simulink model "WindPVStorage_AC_Island"  (R2025a)
settings: Solver=FixedStepDiscrete  StartTime=0.0  StopTime=48  FixedStep=1e-4  RelTol=1e-3
libraries: spsGroundLib x9, spsControlledCurrentSourceLib x6, spsThreePhaseParallelRLCLoadLib x5, spsThreePhaseVIMeasurementLib x5, spsSeriesRLCBranchLib x3, spsControlledVoltageSourceLib x3, spsThreePhaseBreakerLib x3, spspowerguiLib x1
settings Model: Creator=cherrycai  LastModifiedBy=cherrycai
settings DataIOCC: SaveOutput=off  SaveTime=off

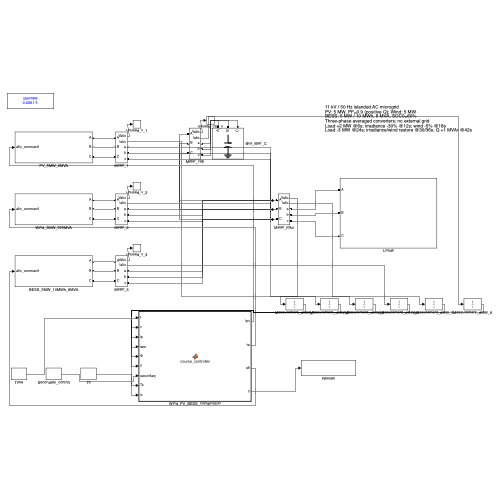
[thumbnail: Simulink's stored preview of the top-level diagram]
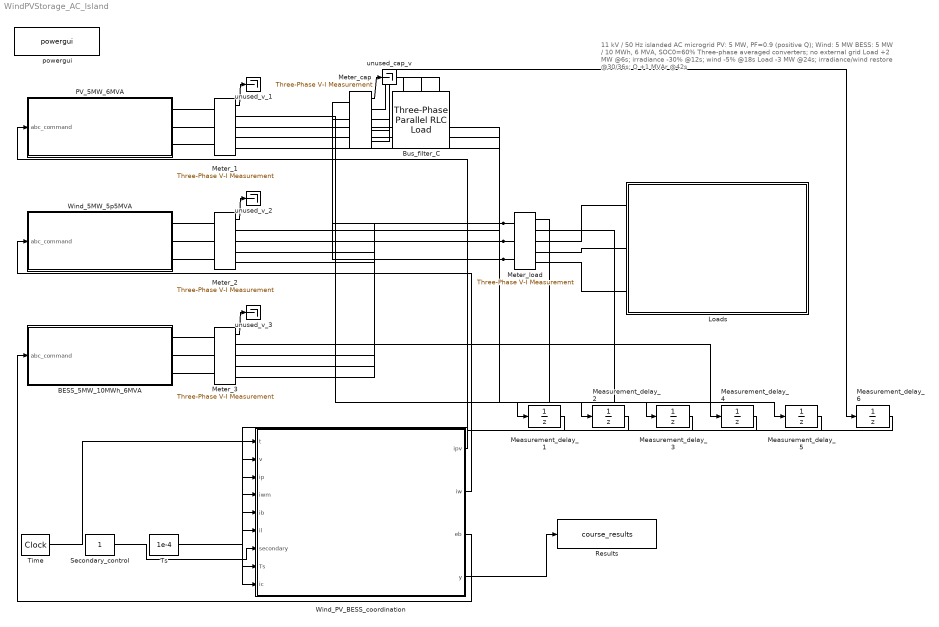
== system WindPVStorage_AC_Island ==
  note: 11 kV / 50 Hz islanded AC microgrid
      | PV: 5 MW, PF=0.9 (positive Q); Wind: 5 MW
      | BESS: 5 MW / 10 MWh, 6 MVA, SOC0=60%
      | Three-phase averaged converters; no external grid
      | Load +2 MW @6s; irradiance -30% @12s; wind -5% @18s
      | Load -3 MW @24s; irradiance/wind restore @30/36s; Q +1 MVAr @42s
  BESS_5MW_10MWh_6MVA : Subsystem
  Bus_filter_C : spsThreePhaseParallelRLCLoadLib/Three-Phase Parallel RLC Load  LConnTagsString=A|B|C  Configuration=Y (grounded)  NominalVoltage=11000  Vabc=[1e3 1e3 1e3]  Vabcp=[1e3 1e3 1e3]  NominalFrequency=50  UnbalancedPower=off  ActivePower=0  InductivePower=0  CapacitivePower=2e5  Pabc=[10e3 9e3 11e3]  QLabc=[100 90 110]  QCabc=[100 90 110]  Pabcp=[10e3 9e3 11e3]  QLabcp=[100 90 110]  QCabcp=[100 90 110]  Measurements=None  LoadType=constant Z
  Loads : Subsystem
  Measurement_delay_{1..6} (6 alike) : UnitDelay  InitialCondition=[0 0 0]  SampleTime=1e-4  HasFrameUpgradeWarning=on
  Meter_1 : spsThreePhaseVIMeasurementLib/Three-Phase V-I Measurement  VoltageMeasurement=phase-to-ground  SetLabelV=off  LabelV=Vabc  Vpu=off  VpuLL=off  CurrentMeasurement=yes  SetLabelI=off  LabelI=Iabc  Ipu=off  Pbase=100e6  Vbase=500e3  OutputType=Complex  PhasorSimulation=off  PSBequivalent=0
  Meter_2 : spsThreePhaseVIMeasurementLib/Three-Phase V-I Measurement  VoltageMeasurement=phase-to-ground  SetLabelV=off  LabelV=Vabc  Vpu=off  VpuLL=off  CurrentMeasurement=yes  SetLabelI=off  LabelI=Iabc  Ipu=off  Pbase=100e6  Vbase=500e3  OutputType=Complex  PhasorSimulation=off  PSBequivalent=0
  Meter_3 : spsThreePhaseVIMeasurementLib/Three-Phase V-I Measurement  VoltageMeasurement=phase-to-ground  SetLabelV=off  LabelV=Vabc  Vpu=off  VpuLL=off  CurrentMeasurement=yes  SetLabelI=off  LabelI=Iabc  Ipu=off  Pbase=100e6  Vbase=500e3  OutputType=Complex  PhasorSimulation=off  PSBequivalent=0
  Meter_cap : spsThreePhaseVIMeasurementLib/Three-Phase V-I Measurement  VoltageMeasurement=phase-to-ground  SetLabelV=off  LabelV=Vabc  Vpu=off  VpuLL=off  CurrentMeasurement=yes  SetLabelI=off  LabelI=Iabc  Ipu=off  Pbase=100e6  Vbase=500e3  OutputType=Complex  PhasorSimulation=off  PSBequivalent=0
  Meter_load : spsThreePhaseVIMeasurementLib/Three-Phase V-I Measurement  VoltageMeasurement=phase-to-ground  SetLabelV=off  LabelV=Vabc  Vpu=off  VpuLL=off  CurrentMeasurement=yes  SetLabelI=off  LabelI=Iabc  Ipu=off  Pbase=100e6  Vbase=500e3  OutputType=Complex  PhasorSimulation=off  PSBequivalent=0
  PV_5MW_6MVA : Subsystem
  Results : ToWorkspace  VariableName=course_results  SaveFormat=Timeseries  SampleTime=-1
      settings: Decimation=10
  Secondary_control : Constant
  Time : DigitalClock  SampleTime=1e-4
  Ts : Constant  Value=1e-4
  Wind_5MW_5p5MVA : Subsystem
  Wind_PV_BESS_coordination : MATLAB Function  TreatAsAtomicUnit=on
  powergui : spspowerguiLib/powergui  Priority=1  SimulationMode=Discrete  SampleTime=1e-4  frequency=50  Iterations=50  frequencyindice=50  Pbase=100e6  ErrMax=1e-4  UnitsV=kV  UnitsW=MW  buscounter=0  FunctionMessages=off  echomessages=off  EnableUseOfTLC=off  CurrentSourceSwitches=off  DisableSnubberDevices=off  DisableRonSwitches=off  DisableVfSwitches=off  DisplayEquations=off  AutomaticDiscreteSolvers=off  SolverType=Tustin/Backward Euler (TBE)  Interpol=off  ExternalGateDelay=off  methode=off  Ts=100  x0status=blocks  SPID=on  SwTol=0  HookPort=off  NonlinearTolerance=1e-4  nMaxIteration=100  ContinueOnMaxIteration=off  RestoreLinks=warning  ResistiveCurrentMeasurement=off  Frange=[0:2:500]  Ylog=off  Xlog=on  ShowGrid=off  save=off  variable=ZData  structure=0  ZoomFFT=off  StartTime=0.0  cycles=1  DisplayStyle=1  fundamental=50  FreqAxis=off  MaxFrequency=1000  frequencyindicesteady=1  RmsSteady=1  display=off
  unused_cap_v : Terminator
  unused_v_1 : Terminator
  unused_v_2 : Terminator
  unused_v_3 : Terminator
  wires:
  Time/1 -> Wind_PV_BESS_coordination/1(t)
  Secondary_control/1 -> Wind_PV_BESS_coordination/7(secondary)
  Ts/1 -> Wind_PV_BESS_coordination/8(Ts)
  Wind_PV_BESS_coordination/1(ipv) -> PV_5MW_6MVA/1(abc_command)
  Wind_PV_BESS_coordination/2(iw) -> Wind_5MW_5p5MVA/1(abc_command)
  Wind_PV_BESS_coordination/3(eb) -> BESS_5MW_10MWh_6MVA/1(abc_command)
  Meter_cap/2 -> Measurement_delay_6/1
  Measurement_delay_6/1 -> Wind_PV_BESS_coordination/9(ic)
  Meter_cap/1 -> unused_cap_v/1
  Meter_load/1 -> Measurement_delay_1/1
  Measurement_delay_1/1 -> Wind_PV_BESS_coordination/2(v)
  Meter_1/2 -> Measurement_delay_2/1
  Measurement_delay_2/1 -> Wind_PV_BESS_coordination/3(ip)
  Meter_2/2 -> Measurement_delay_3/1
  Measurement_delay_3/1 -> Wind_PV_BESS_coordination/4(iwm)
  Meter_3/2 -> Measurement_delay_4/1
  Measurement_delay_4/1 -> Wind_PV_BESS_coordination/5(ib)
  Meter_load/2 -> Measurement_delay_5/1
  Measurement_delay_5/1 -> Wind_PV_BESS_coordination/6(il)
  Wind_PV_BESS_coordination/4(y) -> Results/1
  Meter_1/1 -> unused_v_1/1
  Meter_2/1 -> unused_v_2/1
  Meter_3/1 -> unused_v_3/1
  connections:
  PV_5MW_6MVA/RConn1 -- Meter_1/LConn1
  PV_5MW_6MVA/RConn2 -- Meter_1/LConn2
  PV_5MW_6MVA/RConn3 -- Meter_1/LConn3
  Wind_5MW_5p5MVA/RConn1 -- Meter_2/LConn1
  Wind_5MW_5p5MVA/RConn2 -- Meter_2/LConn2
  Wind_5MW_5p5MVA/RConn3 -- Meter_2/LConn3
  BESS_5MW_10MWh_6MVA/RConn1 -- Meter_3/LConn1
  BESS_5MW_10MWh_6MVA/RConn2 -- Meter_3/LConn2
  BESS_5MW_10MWh_6MVA/RConn3 -- Meter_3/LConn3
  Meter_1/RConn1 -- Meter_2/RConn1 -- Meter_3/RConn1 -- Meter_load/LConn1 -- Meter_cap/LConn1
  Meter_1/RConn2 -- Meter_2/RConn2 -- Meter_3/RConn2 -- Meter_load/LConn2 -- Meter_cap/LConn2
  Meter_1/RConn3 -- Meter_2/RConn3 -- Meter_3/RConn3 -- Meter_load/LConn3 -- Meter_cap/LConn3
  Meter_load/RConn1 -- Loads/LConn1
  Meter_load/RConn2 -- Loads/LConn2
  Meter_load/RConn3 -- Loads/LConn3
  Meter_cap/RConn1 -- Bus_filter_C/LConn1
  Meter_cap/RConn2 -- Bus_filter_C/LConn2
  Meter_cap/RConn3 -- Bus_filter_C/LConn3

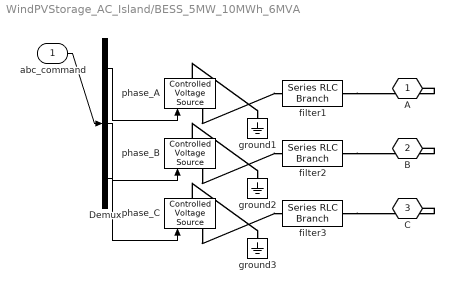
== system WindPVStorage_AC_Island/BESS_5MW_10MWh_6MVA ==
  abc_command : Inport
  Demux : Demux  Outputs=3
  filter1 : spsSeriesRLCBranchLib/Series RLC Branch  LConnTagsString=__new0  RConnTagsString=__new0  BranchType=RL  Resistance=.15  Inductance=.003  SetiL0=off  InitialCurrent=0  Capacitance=1e-6  Setx0=off  InitialVoltage=0  Measurements=None
  filter2 : spsSeriesRLCBranchLib/Series RLC Branch  LConnTagsString=__new0  RConnTagsString=__new0  BranchType=RL  Resistance=.15  Inductance=.003  SetiL0=off  InitialCurrent=0  Capacitance=1e-6  Setx0=off  InitialVoltage=0  Measurements=None
  filter3 : spsSeriesRLCBranchLib/Series RLC Branch  LConnTagsString=__new0  RConnTagsString=__new0  BranchType=RL  Resistance=.15  Inductance=.003  SetiL0=off  InitialCurrent=0  Capacitance=1e-6  Setx0=off  InitialVoltage=0  Measurements=None
  ground1 : spsGroundLib/Ground  LConnTagsString=a
  ground2 : spsGroundLib/Ground  LConnTagsString=a
  ground3 : spsGroundLib/Ground  LConnTagsString=a
  phase_A : spsControlledVoltageSourceLib/Controlled Voltage Source  Initialize=off  Source_Type=AC  Amplitude=0  Phase=0  Frequency=0  Measurements=None
  phase_B : spsControlledVoltageSourceLib/Controlled Voltage Source  Initialize=off  Source_Type=AC  Amplitude=0  Phase=0  Frequency=0  Measurements=None
  phase_C : spsControlledVoltageSourceLib/Controlled Voltage Source  Initialize=off  Source_Type=AC  Amplitude=0  Phase=0  Frequency=0  Measurements=None
  A : PMIOPort  Side=Right
  B : PMIOPort  Port=2  Side=Right
  C : PMIOPort  Port=3  Side=Right
  wires:
  abc_command/1 -> Demux/1
  Demux/1 -> phase_A/1
  Demux/2 -> phase_B/1
  Demux/3 -> phase_C/1
  connections:
  phase_A/RConn1 -- ground1/LConn1
  phase_A/LConn1 -- filter1/LConn1
  filter1/RConn1 -- A/RConn1
  phase_B/RConn1 -- ground2/LConn1
  phase_B/LConn1 -- filter2/LConn1
  filter2/RConn1 -- B/RConn1
  phase_C/RConn1 -- ground3/LConn1
  phase_C/LConn1 -- filter3/LConn1
  filter3/RConn1 -- C/RConn1

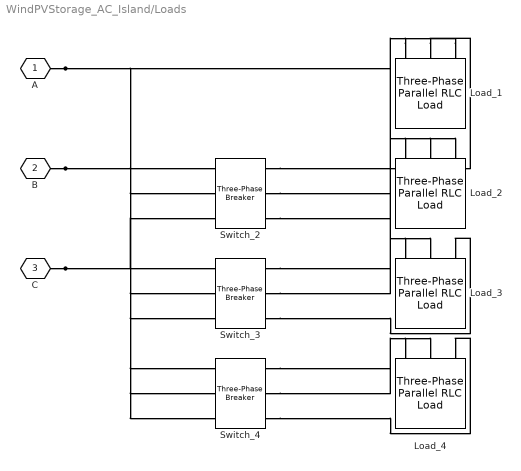
== system WindPVStorage_AC_Island/Loads ==
  Load_1 : spsThreePhaseParallelRLCLoadLib/Three-Phase Parallel RLC Load  LConnTagsString=A|B|C  Configuration=Y (grounded)  NominalVoltage=11000  Vabc=[1e3 1e3 1e3]  Vabcp=[1e3 1e3 1e3]  NominalFrequency=50  UnbalancedPower=off  ActivePower=7000000  InductivePower=2000000  CapacitivePower=0  Pabc=[10e3 9e3 11e3]  QLabc=[100 90 110]  QCabc=[100 90 110]  Pabcp=[10e3 9e3 11e3]  QLabcp=[100 90 110]  QCabcp=[100 90 110]  Measurements=None  LoadType=constant Z
  Load_2 : spsThreePhaseParallelRLCLoadLib/Three-Phase Parallel RLC Load  LConnTagsString=A|B|C  Configuration=Y (grounded)  NominalVoltage=11000  Vabc=[1e3 1e3 1e3]  Vabcp=[1e3 1e3 1e3]  NominalFrequency=50  UnbalancedPower=off  ActivePower=3000000  InductivePower=300000  CapacitivePower=0  Pabc=[10e3 9e3 11e3]  QLabc=[100 90 110]  QCabc=[100 90 110]  Pabcp=[10e3 9e3 11e3]  QLabcp=[100 90 110]  QCabcp=[100 90 110]  Measurements=None  LoadType=constant Z
  Load_3 : spsThreePhaseParallelRLCLoadLib/Three-Phase Parallel RLC Load  LConnTagsString=A|B|C  Configuration=Y (grounded)  NominalVoltage=11000  Vabc=[1e3 1e3 1e3]  Vabcp=[1e3 1e3 1e3]  NominalFrequency=50  UnbalancedPower=off  ActivePower=2000000  InductivePower=200000  CapacitivePower=0  Pabc=[10e3 9e3 11e3]  QLabc=[100 90 110]  QCabc=[100 90 110]  Pabcp=[10e3 9e3 11e3]  QLabcp=[100 90 110]  QCabcp=[100 90 110]  Measurements=None  LoadType=constant Z
  Load_4 : spsThreePhaseParallelRLCLoadLib/Three-Phase Parallel RLC Load  LConnTagsString=A|B|C  Configuration=Y (grounded)  NominalVoltage=11000  Vabc=[1e3 1e3 1e3]  Vabcp=[1e3 1e3 1e3]  NominalFrequency=50  UnbalancedPower=off  ActivePower=0  InductivePower=1000000  CapacitivePower=0  Pabc=[10e3 9e3 11e3]  QLabc=[100 90 110]  QCabc=[100 90 110]  Pabcp=[10e3 9e3 11e3]  QLabcp=[100 90 110]  QCabcp=[100 90 110]  Measurements=None  LoadType=constant Z
  Switch_2 : spsThreePhaseBreakerLib/Three-Phase Breaker  InitialState=closed  SwitchA=on  SwitchB=on  SwitchC=on  SwitchTimes=24  External=off  BreakerResistance=.001  SnubberResistance=1e8  SnubberCapacitance=inf  Measurements=None
  Switch_3 : spsThreePhaseBreakerLib/Three-Phase Breaker  InitialState=open  SwitchA=on  SwitchB=on  SwitchC=on  SwitchTimes=6  External=off  BreakerResistance=.001  SnubberResistance=1e8  SnubberCapacitance=inf  Measurements=None
  Switch_4 : spsThreePhaseBreakerLib/Three-Phase Breaker  InitialState=open  SwitchA=on  SwitchB=on  SwitchC=on  SwitchTimes=42  External=off  BreakerResistance=.001  SnubberResistance=1e8  SnubberCapacitance=inf  Measurements=None
  A : PMIOPort  Side=Left
  B : PMIOPort  Port=2  Side=Left
  C : PMIOPort  Port=3  Side=Left
  connections:
  Load_1/LConn1 -- A/RConn1 -- Switch_2/LConn1 -- Switch_3/LConn1 -- Switch_4/LConn1
  Load_1/LConn2 -- B/RConn1 -- Switch_2/LConn2 -- Switch_3/LConn2 -- Switch_4/LConn2
  Load_1/LConn3 -- C/RConn1 -- Switch_2/LConn3 -- Switch_3/LConn3 -- Switch_4/LConn3
  Switch_2/RConn1 -- Load_2/LConn1
  Switch_2/RConn2 -- Load_2/LConn2
  Switch_2/RConn3 -- Load_2/LConn3
  Switch_3/RConn1 -- Load_3/LConn1
  Switch_3/RConn2 -- Load_3/LConn2
  Switch_3/RConn3 -- Load_3/LConn3
  Switch_4/RConn1 -- Load_4/LConn1
  Switch_4/RConn2 -- Load_4/LConn2
  Switch_4/RConn3 -- Load_4/LConn3

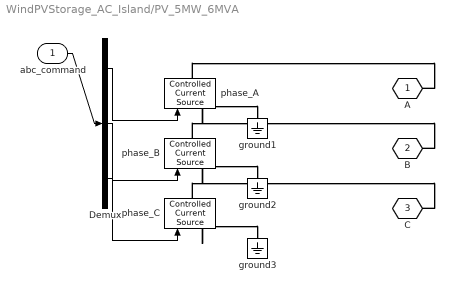
== system WindPVStorage_AC_Island/PV_5MW_6MVA ==
  abc_command : Inport
  Demux : Demux  Outputs=3
  ground1 : spsGroundLib/Ground  LConnTagsString=a
  ground2 : spsGroundLib/Ground  LConnTagsString=a
  ground3 : spsGroundLib/Ground  LConnTagsString=a
  phase_A : spsControlledCurrentSourceLib/Controlled Current Source  Initialize=off  Source_Type=AC  Amplitude=0  Phase=0  Frequency=0  Measurements=None
  phase_B : spsControlledCurrentSourceLib/Controlled Current Source  Initialize=off  Source_Type=AC  Amplitude=0  Phase=0  Frequency=0  Measurements=None
  phase_C : spsControlledCurrentSourceLib/Controlled Current Source  Initialize=off  Source_Type=AC  Amplitude=0  Phase=0  Frequency=0  Measurements=None
  A : PMIOPort  Side=Right
  B : PMIOPort  Port=2  Side=Right
  C : PMIOPort  Port=3  Side=Right
  wires:
  abc_command/1 -> Demux/1
  Demux/1 -> phase_A/1
  Demux/2 -> phase_B/1
  Demux/3 -> phase_C/1
  connections:
  phase_A/LConn1 -- ground1/LConn1
  phase_A/RConn1 -- A/RConn1
  phase_B/LConn1 -- ground2/LConn1
  phase_B/RConn1 -- B/RConn1
  phase_C/LConn1 -- ground3/LConn1
  phase_C/RConn1 -- C/RConn1

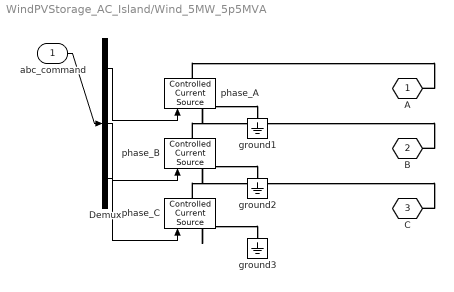
== system WindPVStorage_AC_Island/Wind_5MW_5p5MVA ==
  abc_command : Inport
  Demux : Demux  Outputs=3
  ground1 : spsGroundLib/Ground  LConnTagsString=a
  ground2 : spsGroundLib/Ground  LConnTagsString=a
  ground3 : spsGroundLib/Ground  LConnTagsString=a
  phase_A : spsControlledCurrentSourceLib/Controlled Current Source  Initialize=off  Source_Type=AC  Amplitude=0  Phase=0  Frequency=0  Measurements=None
  phase_B : spsControlledCurrentSourceLib/Controlled Current Source  Initialize=off  Source_Type=AC  Amplitude=0  Phase=0  Frequency=0  Measurements=None
  phase_C : spsControlledCurrentSourceLib/Controlled Current Source  Initialize=off  Source_Type=AC  Amplitude=0  Phase=0  Frequency=0  Measurements=None
  A : PMIOPort  Side=Right
  B : PMIOPort  Port=2  Side=Right
  C : PMIOPort  Port=3  Side=Right
  wires:
  abc_command/1 -> Demux/1
  Demux/1 -> phase_A/1
  Demux/2 -> phase_B/1
  Demux/3 -> phase_C/1
  connections:
  phase_A/LConn1 -- ground1/LConn1
  phase_A/RConn1 -- A/RConn1
  phase_B/LConn1 -- ground2/LConn1
  phase_B/RConn1 -- B/RConn1
  phase_C/LConn1 -- ground3/LConn1
  phase_C/RConn1 -- C/RConn1

== matlab function WindPVStorage_AC_Island/Wind_PV_BESS_coordination ==
  data: ipv output; iw output; eb output; t input; y output; v input; ip input; iwm input; ib input; il input; secondary input; Ts input; ic input
function [ipv,iw,eb,y] = course_controller(t,v,ip,iwm,ib,il,secondary,Ts,ic)
% Three-phase averaged converters. SI units; generation P,Q positive.
% The battery establishes voltage/frequency. PV and wind follow the AC bus.
% Parameters are engineering choices for this course, not manufacturer data.
%#codegen
persistent fp theta ep soc pp pw pref xi uv pfilt qfilt ufilt fm oldangle pc qc wc pll pllint wqc
if isempty(fp)
    fp=50; theta=0; ep=1; soc=.60; pp=5e6; pw=5e6;
    pref=0; xi=0; uv=0; pfilt=0; qfilt=0; ufilt=1;
    fm=50; oldangle=0; pc=0; qc=0; wc=0; pll=0;pllint=0;wqc=0;
end
Vpk=11000*sqrt(2/3); kq=sqrt(1/.9^2-1);
[Pp,Qp]=pq(v,ip); [Pw,Qw]=pq(v,iwm);
[Pb,Qb]=pq(v,ib); [Pl,Ql]=pq(v,il);
[Pcap,Qcap]=pq(v,ic);
va=(2*v(1)-v(2)-v(3))/3; vb=(v(2)-v(3))/sqrt(3);
vm=sqrt(va*va+vb*vb); u=vm/Vpk; ang=atan2(vb,va);
delta=atan2(sin(ang-oldangle),cos(ang-oldangle)); oldangle=ang;
if u>.4 && t>.1, fm=fm+Ts/.04*(delta/(2*pi*Ts)-fm); end
ufilt=ufilt+Ts/.02*(u-ufilt);
pfilt=pfilt+Ts/.02*(Pb-pfilt); qfilt=qfilt+Ts/.02*(Qb-qfilt);
pllerr=(-va*sin(pll)+vb*cos(pll))/max(Vpk*ufilt,.2*Vpk);
pllint=lim(pllint+Ts*4000*pllerr,-20*pi,20*pi);
wpll=2*pi*50+120*pllerr+pllint;

% Irradiance and wind experiments; nameplate active power is 5 MW each.
G=1000; if t>=12 && t<30, G=700; end
wind=12; if t>=18 && t<36, wind=11.4; end
pav=min(5e6,5e6*G/1000);
wav=min(5e6,5e6*(wind/12)^3);
pp=pp+Ts/.06*(pav-pp); pw=pw+Ts/.30*(wav-pw);
% Slow terminal-power correction compensates discrete synchronous sampling.
if t>1 && u>.8
    pc=lim(pc+Ts*5*(pp-Pp),-.15e6,.15e6);
    qc=lim(qc+Ts*8*(kq*Pp-Qp),-.3e6,.3e6);
    wc=lim(wc+Ts*5*(pw-Pw),-.15e6,.15e6);
    wqc=lim(wqc-Ts*8*Qw,-.3e6,.3e6);
end
pcommand=max(0,pp+pc); qcommand=kq*pp+qc;
scale=min(1,6e6/max(sqrt(pcommand^2+qcommand^2),1));
pcommand=pcommand*scale; qcommand=qcommand*scale;
phase=pll+wpll*Ts; ph=[phase;phase-2*pi/3;phase+2*pi/3];
pll=mod(pll+wpll*Ts,2*pi);
den=max(ufilt,.8)*Vpk; lowvoltage=min(max(ufilt/.8,0),1)*min(t/.25,1)^2;
ipv=2/(3*den)*(pcommand*cos(ph)+qcommand*sin(ph))*lowvoltage;
iw=2/(3*den)*(max(0,pw+wc)*cos(ph)+wqc*sin(ph))*lowvoltage;
% Two percent current margin covers the small startup voltage overshoot.
ipv=ipv*min(1,(.98*6e6/(sqrt(3)*11000))/max(norm(ipv)/sqrt(3),1));
iw=iw*min(1,(5.5e6/(sqrt(3)*11000))/max(norm(iw)/sqrt(3),1));

% Secondary coordination: measured residual demand feedforward plus f/V PI.
if secondary>.5 && t>1
    xi=lim(xi+Ts*1e6*(50-fm),-1e6,1e6);
    ptarget=lim(Pl-Pp-Pw+xi,-5e6,5e6);
    pref=pref+Ts/.15*(ptarget-pref);
    uv=lim(uv+Ts*.8*(1-ufilt),-.15,.15);
else
    pref=0; xi=0; uv=0;
end
% VSG swing equation, H=2 s, Sbase=6 MVA; 0.5 Hz/5 MW primary droop.
fp=fp+Ts*50/(2*2*6e6)*(pref-pfilt-10e6*(fp-50));
etarget=lim(1+uv-.02*qfilt/1e6,.85,1.15);
ep=ep+Ts/.05*(etarget-ep);
phb=[theta;theta-2*pi/3;theta+2*pi/3];
ib_rms=norm(ib)/sqrt(3); Imax=6e6/(sqrt(3)*11000);
% Extra virtual resistance only above 1.15 pu current; not active in tests.
rv=lim((ib_rms/Imax-1.15)*10,0,3);
eb=Vpk*ep*min(t/.25,1)*cos(phb)-rv*ib;
theta=mod(theta+2*pi*fp*Ts,2*pi);
% Battery energy includes series-resistance losses and 96% efficiency.
pdc=Pb+3*.15*ib_rms^2;
if pdc>=0, de=pdc/.96; else, de=pdc*.96; end
soc=soc-Ts*de/(10e6*3600);
PF=abs(Pp)/max(sqrt(Pp^2+Qp^2),1);
y=[Pp;Qp;Pw;Qw;Pb;Qb;Pl;Ql;fm;u;fp;soc;PF;pref;ep;G;wind;pav;wav;ib_rms;norm(ip)/sqrt(3);norm(iwm)/sqrt(3);Pp+Pw+Pb-Pl-Pcap;Qp+Qw+Qb-Ql-Qcap;pdc;double(rv>0);v;ip;ib;Pcap;Qcap];
end
function [P,Q]=pq(v,i)
va=(2*v(1)-v(2)-v(3))/3; vb=(v(2)-v(3))/sqrt(3);
ia=(2*i(1)-i(2)-i(3))/3; ib=(i(2)-i(3))/sqrt(3);
P=dot(v,i); Q=1.5*(vb*ia-va*ib);
end
function y=lim(x,a,b)
y=min(max(x,a),b);
end
